simulink model "fully_actuated_manipulator"  (R2025b)
settings: Solver=VariableStepAuto  StartTime=0.0  StopTime=20  RelTol=1e-3
settings Model: Creator=Vishrut  LastModifiedBy=Vishrut

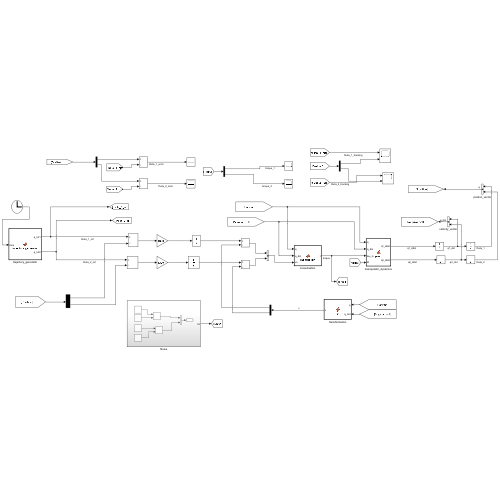
[thumbnail: Simulink's stored preview of the top-level diagram]
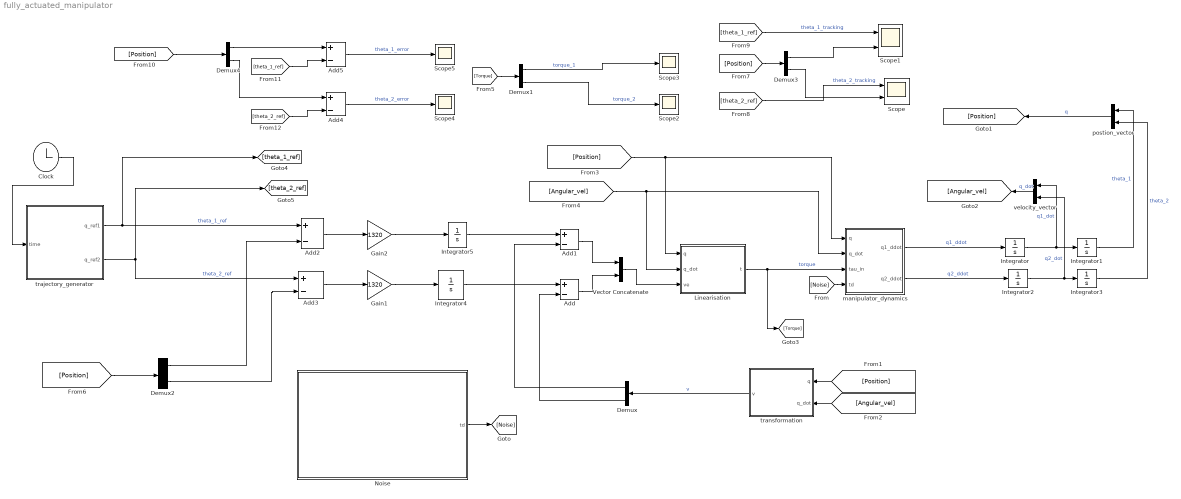
== system fully_actuated_manipulator ==
  Add{,1..5} (6 alike) : Sum  Inputs=+-
  Clock : Clock
  Demux{,1..4} (5 alike) : Demux  Outputs=2
  Gain1 : Gain  Gain=1320
  Gain2 : Gain  Gain=1320
  Integrator{,2,4..5} (4 alike) : Integrator
  Integrator1 : Integrator  InitialCondition=1.0
  Integrator3 : Integrator  InitialCondition=1.5
  Linearisation : MATLAB Function  TreatAsAtomicUnit=on
  Noise : Subsystem
  Scope : Scope  NumInputPorts=2
      settings: ActiveDisplayYMinimum=0.73660737474858073  ActiveDisplayYMaximum=2.4082480556569132
  Scope1 : Scope  NumInputPorts=2
      settings: ActiveDisplayYMinimum=-1  ActiveDisplayYMaximum=1
  Scope{2..5} (4 alike) : Scope
      Scope2 settings: DataLoggingVariableName=ScopeData2
      Scope3 settings: DataLoggingVariableName=ScopeData3
      Scope4 settings: ActiveDisplayYMinimum=-1  ActiveDisplayYMaximum=1  DataLoggingVariableName=ScopeData4
      Scope5 settings: ActiveDisplayYMinimum=-1  ActiveDisplayYMaximum=1  DataLoggingVariableName=ScopeData5
  Vector Concatenate : Concatenate
  manipulator_dynamics : MATLAB Function  TreatAsAtomicUnit=on
  postion_vector : Concatenate
  trajectory_generator : MATLAB Function  TreatAsAtomicUnit=on
  transformation : MATLAB Function  TreatAsAtomicUnit=on
  velocity_vector : Concatenate
  wires:
  manipulator_dynamics/1(q1_ddot) -> Integrator/1  "q1_ddot"
  manipulator_dynamics/2(q2_ddot) -> Integrator2/1  "q2_ddot"
  Add1/1 -> Vector Concatenate/1
  Add/1 -> Vector Concatenate/2
  Clock/1 -> trajectory_generator/1(time)
  Add2/1 -> Gain2/1
  Integrator5/1 -> Add1/1
  trajectory_generator/1(q_ref1) -> Add2/1, [theta_1_ref]  "theta_1_ref"
  trajectory_generator/2(q_ref2) -> Add3/1, [theta_2_ref]  "theta_2_ref"
  Add3/1 -> Gain1/1
  Gain1/1 -> Integrator4/1
  Integrator4/1 -> Add/1
  transformation/1(v) -> Demux/1  "v"
  Add4/1 -> Scope4/1  "theta_2_error"
  Demux1/1 -> Scope3/1  "torque_1"
  Demux1/2 -> Scope2/1  "torque_2"
  Add5/1 -> Scope5/1  "theta_1_error"
  Gain2/1 -> Integrator5/1
  Linearisation/1(t) -> [Torque], manipulator_dynamics/3(tau_in)  "torque"
  Vector Concatenate/1 -> Linearisation/3(ve)
  Integrator2/1 -> velocity_vector/2, Integrator3/1  "q2_dot"
  Integrator/1 -> velocity_vector/1, Integrator1/1  "q1_dot"
  Integrator1/1 -> postion_vector/1  "theta_1"
  Integrator3/1 -> postion_vector/2  "theta_2"
  Demux/1 -> Add1/2
  Demux/2 -> Add/2
  Noise/1(td) -> [Noise]
  postion_vector/1 -> [Position]  "q"
  velocity_vector/1 -> [Angular_vel]  "q_dot"
  [Position] -> transformation/1(q)
  [Angular_vel] -> transformation/2(q_dot)
  [Angular_vel] -> Linearisation/2(q_dot), manipulator_dynamics/2(q_dot)
  [Position] -> Linearisation/1(q), manipulator_dynamics/1(q)
  [Torque] -> Demux1/1
  [Position] -> Demux2/1
  Demux2/1 -> Add2/2
  Demux2/2 -> Add3/2
  [Position] -> Demux3/1
  Demux3/1 -> Scope1/2
  [theta_1_ref] -> Scope1/1  "theta_1_tracking"
  [Position] -> Demux4/1
  Demux4/1 -> Add5/1
  Demux4/2 -> Add4/1
  [theta_1_ref] -> Add5/2
  [theta_2_ref] -> Add4/2
  [theta_2_ref] -> Scope/1  "theta_2_tracking"
  Demux3/2 -> Scope/2
  [Noise] -> manipulator_dynamics/4(td)

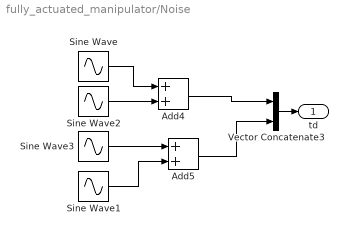
== system fully_actuated_manipulator/Noise ==
  Add4 : Sum
  Add5 : Sum
  Sine Wave : Sin  Amplitude=2  SampleTime=0
  Sine Wave1 : Sin  Frequency=2  Phase=pi/2  SampleTime=0
  Sine Wave2 : Sin  Amplitude=0.5  Frequency=200*pi  SampleTime=0
  Sine Wave3 : Sin  Amplitude=0.5  Frequency=200*pi  SampleTime=0
  Vector Concatenate3 : Concatenate
  td : Outport
  wires:
  Add4/1 -> Vector Concatenate3/1
  Add5/1 -> Vector Concatenate3/2
  Sine Wave3/1 -> Add5/1
  Sine Wave/1 -> Add4/1
  Sine Wave2/1 -> Add4/2
  Vector Concatenate3/1 -> td/1
  Sine Wave1/1 -> Add5/2

== matlab function fully_actuated_manipulator/Linearisation ==
  data: q input size=[2 1]; q_dot input size=[2 1]; ve input size=[2 1]; t output size=[2 1]
function t = linearisation(q,q_dot,ve)


l1 = 1; l2 = 0.8; m1 = 0.5; m2 = 1.5;
j1 = 5; j2 = 5; g = 9.8;

 m11 = m1*l1^2 + m2*(l1^2 + l2^2 + 2*l1*l2*cos(q(2))) + j1 + j2;
 m12 = m2*(l1*l2*cos(q(2)) + l2^2) + j2;
 m21 = m12;
 m22 = m2*l2^2 + j2;
 M = [m11, m12; m21, m22];
 
 h_val = m2*l1*l2*sin(q(2));
 C_vec = [-h_val*q_dot(2)^2 - 2*h_val*q_dot(1)*q_dot(2); 
              h_val*q_dot(1)^2];

  G1 = (m1 + m2)*l1*g*cos(q(1)) + m2*g*l2*cos(q(1) + q(2));
  G2 = m2*g*l2*cos(q(1) + q(2));
  G_vec = [G1; G2];

  t = M * ve + C_vec + G_vec;

end

== matlab function fully_actuated_manipulator/manipulator_dynamics ==
  data: q input size=[2 1]; q_dot input size=[2 1]; tau_in input size=[2 1]; q1_ddot output; q2_ddot output; td input size=[2 1]
function [q1_ddot, q2_ddot] = plant(q, q_dot, tau_in,td)


l1 = 1; l2 = 0.8; 
m1 = 0.5; m2 = 1.5;
j1 = 5; j2 = 5; 
g = 9.8;

m11 = m1*l1^2 + m2*(l1^2 + l2^2 + 2*l1*l2*cos(q(2))) + j1 + j2;
m12 = m2*(l2^2 + l1*l2*cos(q(2))) + j2;
m21 = m12;
m22 = m2*l2^2 + j2;
M = [m11, m12; m21, m22];

h = m2*l1*l2*sin(q(2));
C_vec = [-h*q_dot(2)^2 - 2*h*q_dot(1)*q_dot(2); 
          h*q_dot(1)^2];

G1 = (m1 + m2)*l1*g*cos(q(1)) + m2*l2*g*cos(q(1) + q(2));
G2 = m2*l2*g*cos(q(1) + q(2));
G_vec = [G1; G2];

td = [0;0];

q2 = M \ (tau_in + td - C_vec - G_vec);

q1_ddot = q2(1);
q2_ddot = q2(2);

end

== matlab function fully_actuated_manipulator/trajectory_generator ==
  data: time input; q_ref1 output; q_ref2 output
function [q_ref1,q_ref2] = trajectory_generator(time)


q_ref1 = 1.25 - (7/5)*exp(-time) + (7/20)*exp(-4*time);

q_ref2 = 1.25 + exp(-time) - (1/4)*exp(-4*time);





end

== matlab function fully_actuated_manipulator/transformation ==
  data: q input size=[2 1]; v output size=[2 1]; q_dot input size=[2 1]
function v = fcn(q, q_dot)


kp = 362;                       
kd = 33;                            
z1 = q;
z2 = q_dot;
v_pos = kp * z1;
v_vel = kd * z2;
v = v_pos + v_vel;

end
